simulink library "WECSim_Lib_Body_Elements"  (R2020b)
settings: Solver=VariableStepAuto  StartTime=0.0  StopTime=10.0  RelTol=1e-3
undefined symbols (not defined in the file or in its folder): body, simu, waves, X, Y, Z
libraries: nesl_utility x22, sm_lib x16, $bdroot x9, vrlib x3
(part 5 of 5)

== system WECSim_Lib_Body_Elements/Rigid Body/Hydrodynamic Body/Morison Element and Viscous Damping Force Calculation/Morison Element Variant Subsystem/Morison Element On/Regular Wave Morison Force ==
  displacement : Inport
  velocity : Inport  Port=2
  acceleration : Inport  Port=3
  time : Inport  Port=4
  Area : Constant  Value=body.morisonElement.area  VectorParams1D=off
  Ca : Constant  Value=body.morisonElement.ca  VectorParams1D=off
  Cd : Constant  Value=body.morisonElement.cd  VectorParams1D=off
  Current Depth : Constant  Value=waves.current.depth
  Current Direction : Constant  Value=waves.current.direction
  Current Option : Constant  Value=waves.current.option
  Current Speed : Constant  Value=waves.current.speed
  Density : Constant  Value=simu.rho
  Gravity : Constant  Value=simu.gravity
  MATLAB Function : MATLAB Function  TreatAsAtomicUnit=on
  Morison Element Option : Constant  Value=body.morisonElement.option
  Ramp Function Time : Constant  Value=simu.rampTime
  Volume : Constant  Value=body.morisonElement.VME  VectorParams1D=off
  WaterDepth : Constant  Value=waves.waterDepth
  WaveAmp : Constant  Value=waves.amplitude
  WaveFreq : Constant  Value=waves.omega
  WaveHeading : Constant  Value=waves.direction
  WaveNumber : Constant  Value=waves.wavenumber
  "r_{g}" : Constant  Value=body.morisonElement.rgME  VectorParams1D=off
  z : Constant  Value=body.morisonElement.z  VectorParams1D=off
  morison_force : Outport
  wires:
  MATLAB Function/1(f) -> morison_force/1
  z/1 -> MATLAB Function/1(z)
  Morison Element Option/1 -> MATLAB Function/23(simuMorison)
  Volume/1 -> MATLAB Function/8(Vol)
  velocity/1 -> MATLAB Function/3(Vel)
  Ramp Function Time/1 -> MATLAB Function/17(rampTime)
  "r_{g}"/1 -> MATLAB Function/2(r)
  time/1 -> MATLAB Function/10(Time)
  Current Depth/1 -> MATLAB Function/21(currentDepth)
  Current Option/1 -> MATLAB Function/22(currentOption)
  displacement/1 -> MATLAB Function/5(Disp)
  Cd/1 -> MATLAB Function/7(Cd)
  WaveFreq/1 -> MATLAB Function/15(w)
  WaveHeading/1 -> MATLAB Function/12(waveDir)
  Density/1 -> MATLAB Function/11(rho)
  acceleration/1 -> MATLAB Function/4(Accel)
  WaterDepth/1 -> MATLAB Function/13(waterDepth)
  Area/1 -> MATLAB Function/6(Area)
  Current Direction/1 -> MATLAB Function/20(currentDirection)
  Ca/1 -> MATLAB Function/9(Ca)
  WaveNumber/1 -> MATLAB Function/14(k)
  Gravity/1 -> MATLAB Function/18(g)
  WaveAmp/1 -> MATLAB Function/16(A)
  Current Speed/1 -> MATLAB Function/19(currentSpeed)

== system WECSim_Lib_Body_Elements/Rigid Body/Hydrodynamic Body/Wave Radiation Forces Calculation/SS CI and Constant-Damping-CoeVariant Subsystem/Convolution Integral Calculation/Convolution Variant Subsystem ==
  velocity : Inport
  Convolution Integral Calculation : Subsystem  VariantControl=sv_b1_noVariableHydro
  Convolution Integral Surface Calculation : Subsystem  VariantControl=sv_b1_variableHydro
  Frad : Outport

== system WECSim_Lib_Body_Elements/Rigid Body/Hydrodynamic Body/Wave Radiation Forces Calculation/SS CI and Constant-Damping-CoeVariant Subsystem/FIR Filter Calculation/FIR Filter Matrix ==
  velocity : Inport
  FIR_filter_row : Subsystem  mask{body=body, B2B=simu.b2b, rowNo=1}
      mask prompts: body "BodyClass"
      mask init: same as WECSim_Lib_Body_Elements/Flex Body/Wave Radiation Forces Calculation/Wave Radiation Forces Calculation/SS CI and Constant-Damping-CoeVariant Subsystem/FIR Filter Calculation/FIR Filter Matrix/FIR_filter_row
  Gain : Gain  Gain=simu.cicDt
  Mux : Mux  Inputs=1
  Out1 : Outport
  wires:
  Mux/1 -> Gain/1
  velocity/1 -> FIR_filter_row/1(In1)
  FIR_filter_row/1(Out1) -> Mux/1
  Gain/1 -> Out1/1

== system WECSim_Lib_Body_Elements/Flex Body/Wave Radiation Forces Calculation/Wave Radiation Forces Calculation/SS CI and Constant-Damping-CoeVariant Subsystem/Convolution Integral Calculation/Convolution Variant Subsystem/Convolution Integral Calculation ==
  note: Calculate the convolution integral using the radiation IRF (body.hydroForce.irkb) and the velocity.
  velocity : Inport
  Bus Selector : BusSelector  OutputSignals=irkb
  MATLAB Function : MATLAB Function  TreatAsAtomicUnit=on
  MATLAB Function1 : MATLAB Function  TreatAsAtomicUnit=on  SystemSampleTime=simu.cicDt
  Rate Transition : RateTransition  InitialCondition=simu.cicDt*[-1 -2 -3]
  Rate Transition1 : RateTransition
  cicTime : Constant  Value=simu.cicTime
  Frad : Outport
  wires:
  MATLAB Function1/2(FradExtrap) -> Rate Transition1/1
  MATLAB Function1/1(timeExtrap) -> Rate Transition/1
  Rate Transition/1 -> MATLAB Function/1(timeExtrap)
  Rate Transition1/1 -> MATLAB Function/2(FradExtrap)
  MATLAB Function/1(Frad) -> Frad/1
  [Clock] -> MATLAB Function1/4(time), MATLAB Function/3(time)
  velocity/1 -> MATLAB Function1/1(velocity)
  [body1_hydroForce] -> Bus Selector/1
  Bus Selector/1 -> MATLAB Function1/2(IRKB)  "<irkb>"
  cicTime/1 -> MATLAB Function1/3(cicTime)

== system WECSim_Lib_Body_Elements/Flex Body/Wave Radiation Forces Calculation/Wave Radiation Forces Calculation/SS CI and Constant-Damping-CoeVariant Subsystem/Convolution Integral Calculation/Convolution Variant Subsystem/Convolution Integral Surface Calculation ==
  note: Calculate the convolution integral using the radiation IRF surface (body.variableHydro.radiationIrfSurface) and the velocity.
  velocity : Inport
  MATLAB Function : MATLAB Function  TreatAsAtomicUnit=on
  Rate Transition : RateTransition  InitialCondition=simu.cicDt*[-1 -2 -3]
  Rate Transition1 : RateTransition
  cicTime : Constant  Value=simu.cicTime
  convolutionIntegralSurface : MATLAB Function  TreatAsAtomicUnit=on  SystemSampleTime=simu.cicDt
  hydroForceIndexInitial : Constant  Value=body.variableHydro.hydroForceIndexInitial
  radiationIrfSurface : Constant  Value=body.variableHydro.radiationIrfSurface
  Frad : Outport
  wires:
  Rate Transition/1 -> MATLAB Function/1(timeExtrap)
  Rate Transition1/1 -> MATLAB Function/2(FradExtrap)
  convolutionIntegralSurface/1(timeExtrap) -> Rate Transition/1
  convolutionIntegralSurface/2(FradExtrap) -> Rate Transition1/1
  MATLAB Function/1(Frad) -> Frad/1
  [Clock] -> convolutionIntegralSurface/6(time), MATLAB Function/3(time)
  [body1_hydroForce] -> convolutionIntegralSurface/2(hydroForceIndex)
  hydroForceIndexInitial/1 -> convolutionIntegralSurface/3(hydroForceIndexInitial)
  radiationIrfSurface/1 -> convolutionIntegralSurface/4(irkbSurfaceInput)
  cicTime/1 -> convolutionIntegralSurface/5(cicTime)
  velocity/1 -> convolutionIntegralSurface/1(velocity)

== system WECSim_Lib_Body_Elements/Flex Body/Wave Radiation Forces Calculation/Wave Radiation Forces Calculation/SS CI and Constant-Damping-CoeVariant Subsystem/FIR Filter Calculation/FIR Filter Matrix/FIR_filter_row ==
  In1 : Inport
  Add : Sum  Inputs=++++++
  Demux : Demux  Outputs=6
      settings: AttributesFormatString=%<Outputs>
  Discrete FIR Filter : DiscreteFir  Coefficients=transpose(squeeze(body.hydroForce.hf1.irkb(:,1,1)))
  Discrete FIR Filter 2 : DiscreteFir  Coefficients=transpose(squeeze(body.hydroForce.hf1.irkb(:,1,2)))
  Discrete FIR Filter 3 : DiscreteFir  Coefficients=transpose(squeeze(body.hydroForce.hf1.irkb(:,1,3)))
  Discrete FIR Filter 4 : DiscreteFir  Coefficients=transpose(squeeze(body.hydroForce.hf1.irkb(:,1,4)))
  Discrete FIR Filter 5 : DiscreteFir  Coefficients=transpose(squeeze(body.hydroForce.hf1.irkb(:,1,5)))
  Discrete FIR Filter 6 : DiscreteFir  Coefficients=transpose(squeeze(body.hydroForce.hf1.irkb(:,1,6)))
  Out1 : Outport
  wires:
  Discrete FIR Filter 6/1 -> Add/6
  Demux/6 -> Discrete FIR Filter 6/1
  Discrete FIR Filter 5/1 -> Add/5
  Demux/5 -> Discrete FIR Filter 5/1
  Discrete FIR Filter 4/1 -> Add/4
  Demux/4 -> Discrete FIR Filter 4/1
  Discrete FIR Filter 3/1 -> Add/3
  Demux/3 -> Discrete FIR Filter 3/1
  Discrete FIR Filter 2/1 -> Add/2
  Demux/2 -> Discrete FIR Filter 2/1
  Discrete FIR Filter/1 -> Add/1
  Demux/1 -> Discrete FIR Filter/1
  Add/1 -> Out1/1
  In1/1 -> Demux/1

== system WECSim_Lib_Body_Elements/Rigid Body/Hydrodynamic Body/Wave Radiation Forces Calculation/SS CI and Constant-Damping-CoeVariant Subsystem/Convolution Integral Calculation/Convolution Variant Subsystem/Convolution Integral Calculation ==
  note: Calculate the convolution integral using the radiation IRF (body.hydroForce.irkb) and the velocity.
  velocity : Inport
  Bus Selector : BusSelector  OutputSignals=irkb
  MATLAB Function : MATLAB Function  TreatAsAtomicUnit=on
  MATLAB Function1 : MATLAB Function  TreatAsAtomicUnit=on  SystemSampleTime=simu.cicDt
  Rate Transition : RateTransition  InitialCondition=simu.cicDt*[-1 -2 -3]
  Rate Transition1 : RateTransition
  cicTime : Constant  Value=simu.cicTime
  Frad : Outport
  wires:
  cicTime/1 -> MATLAB Function1/3(cicTime)
  Bus Selector/1 -> MATLAB Function1/2(IRKB)  "<irkb>"
  [body1_hydroForce] -> Bus Selector/1
  velocity/1 -> MATLAB Function1/1(velocity)
  [Clock] -> MATLAB Function/3(time), MATLAB Function1/4(time)
  MATLAB Function/1(Frad) -> Frad/1
  Rate Transition1/1 -> MATLAB Function/2(FradExtrap)
  Rate Transition/1 -> MATLAB Function/1(timeExtrap)
  MATLAB Function1/1(timeExtrap) -> Rate Transition/1
  MATLAB Function1/2(FradExtrap) -> Rate Transition1/1

== system WECSim_Lib_Body_Elements/Rigid Body/Hydrodynamic Body/Wave Radiation Forces Calculation/SS CI and Constant-Damping-CoeVariant Subsystem/Convolution Integral Calculation/Convolution Variant Subsystem/Convolution Integral Surface Calculation ==
  note: Calculate the convolution integral using the radiation IRF surface (body.variableHydro.radiationIrfSurface) and the velocity.
  velocity : Inport
  MATLAB Function : MATLAB Function  TreatAsAtomicUnit=on
  Rate Transition : RateTransition  InitialCondition=simu.cicDt*[-1 -2 -3]
  Rate Transition1 : RateTransition
  cicTime : Constant  Value=simu.cicTime
  convolutionIntegralSurface : MATLAB Function  TreatAsAtomicUnit=on  SystemSampleTime=simu.cicDt
  hydroForceIndexInitial : Constant  Value=body.variableHydro.hydroForceIndexInitial
  radiationIrfSurface : Constant  Value=body.variableHydro.radiationIrfSurface
  Frad : Outport
  wires:
  velocity/1 -> convolutionIntegralSurface/1(velocity)
  cicTime/1 -> convolutionIntegralSurface/5(cicTime)
  radiationIrfSurface/1 -> convolutionIntegralSurface/4(irkbSurfaceInput)
  hydroForceIndexInitial/1 -> convolutionIntegralSurface/3(hydroForceIndexInitial)
  [body1_hydroForceIndex] -> convolutionIntegralSurface/2(hydroForceIndex)
  [Clock] -> MATLAB Function/3(time), convolutionIntegralSurface/6(time)
  MATLAB Function/1(Frad) -> Frad/1
  convolutionIntegralSurface/2(FradExtrap) -> Rate Transition1/1
  convolutionIntegralSurface/1(timeExtrap) -> Rate Transition/1
  Rate Transition1/1 -> MATLAB Function/2(FradExtrap)
  Rate Transition/1 -> MATLAB Function/1(timeExtrap)

== system WECSim_Lib_Body_Elements/Rigid Body/Hydrodynamic Body/Wave Radiation Forces Calculation/SS CI and Constant-Damping-CoeVariant Subsystem/FIR Filter Calculation/FIR Filter Matrix/FIR_filter_row ==
  In1 : Inport
  Add : Sum  Inputs=++++++
  Demux : Demux  Outputs=6
      settings: AttributesFormatString=%<Outputs>
  Discrete FIR Filter : DiscreteFir  Coefficients=transpose(squeeze(body.hydroForce.hf1.irkb(:,1,1)))
  Discrete FIR Filter 2 : DiscreteFir  Coefficients=transpose(squeeze(body.hydroForce.hf1.irkb(:,1,2)))
  Discrete FIR Filter 3 : DiscreteFir  Coefficients=transpose(squeeze(body.hydroForce.hf1.irkb(:,1,3)))
  Discrete FIR Filter 4 : DiscreteFir  Coefficients=transpose(squeeze(body.hydroForce.hf1.irkb(:,1,4)))
  Discrete FIR Filter 5 : DiscreteFir  Coefficients=transpose(squeeze(body.hydroForce.hf1.irkb(:,1,5)))
  Discrete FIR Filter 6 : DiscreteFir  Coefficients=transpose(squeeze(body.hydroForce.hf1.irkb(:,1,6)))
  Out1 : Outport
  wires:
  In1/1 -> Demux/1
  Add/1 -> Out1/1
  Demux/1 -> Discrete FIR Filter/1
  Discrete FIR Filter/1 -> Add/1
  Demux/2 -> Discrete FIR Filter 2/1
  Discrete FIR Filter 2/1 -> Add/2
  Demux/3 -> Discrete FIR Filter 3/1
  Discrete FIR Filter 3/1 -> Add/3
  Demux/4 -> Discrete FIR Filter 4/1
  Discrete FIR Filter 4/1 -> Add/4
  Demux/5 -> Discrete FIR Filter 5/1
  Discrete FIR Filter 5/1 -> Add/5
  Demux/6 -> Discrete FIR Filter 6/1
  Discrete FIR Filter 6/1 -> Add/6

== matlab function WECSim_Lib_Body_Elements/Rigid Body/Hydrodynamic Body/Morison Element and Viscous Damping Force Calculation/Morison Element Variant Subsystem/Morison Element On/No Wave Morison Force/MorisonElement(s) ==
  data: z input; f output; r input; Vel input; Accel input; Disp input; Area input; Cd input; Vol input; Ca input; Time input; rho input; rampTime input; currentSpeed input; currentDirection input; currentDepth input; currentOption input; bodyMorison input
function f = noWaveMorison(z,r,Vel,Accel,Disp,Area,Cd,Vol,Ca,Time,rho,rampTime,currentSpeed,currentDirection,currentDepth,currentOption,bodyMorison)

f = noWaveMorison(z,r,Vel,Accel,Disp,Area,Cd,Vol,Ca,Time,rho,rampTime,currentSpeed,currentDirection,currentDepth,currentOption,bodyMorison);

end

== matlab function WECSim_Lib_Body_Elements/Rigid Body/Hydrodynamic Body/Morison Element and Viscous Damping Force Calculation/Morison Element Variant Subsystem/Morison Element On/Irregular Wave Morison Force/MATLAB Function ==
  data: z input; f output; r input; Vel input; Accel input; Disp input; Area input; Cd input; Vol input; Ca input; Time input; rho input; waveDir input; waveSpread input; waterDepth input; k input; w input; A input; rampTime input; g input; randPhase input; dw input; currentSpeed input; currentDirection input; currentDepth input; currentOption input; simuMorison input
function f = irregWaveMorison(z,r,Vel,Accel,Disp,Area,Cd,Vol,Ca,Time,rho,waveDir,waveSpread,waterDepth,k,w,A,rampTime,g,randPhase,dw,currentSpeed,currentDirection,currentDepth,currentOption,simuMorison)

f = irregWaveMorison(z,r,Vel,Accel,Disp,Area,Cd,Vol,Ca,Time,rho,waveDir,waveSpread,waterDepth,k,w,A,rampTime,g,randPhase,dw,currentSpeed,currentDirection,currentDepth,currentOption,simuMorison);

end

== matlab function WECSim_Lib_Body_Elements/Rigid Body/Hydrodynamic Body/Wave Diffraction and Excitation Force Calculation/Linear Wave Excitation Force Variant Subsystem/Irregular Wave Excitation Force/MATLAB Function2 ==
  data: disp input; dispPhase output; enable input; frequency input; wavenumber input; direction input
function dispPhase  = calcDispPhase(disp, enable, frequency, wavenumber, direction)
% initialize
dispPhase = zeros(length(frequency),length(direction));
% execute
dispPhase = calcDispPhase(disp, enable, direction, frequency, wavenumber);

end

== matlab function WECSim_Lib_Body_Elements/Rigid Body/Hydrodynamic Body/Wave Diffraction and Excitation Force Calculation/Linear Wave Excitation Force Variant Subsystem/Regular Wave NonLinear Yaw/MATLAB Function3 ==
  data: disp input; dispPhase output; enable input; frequency input; wavenumber input; direction input
function dispPhase  = calcDispPhase(disp, enable, frequency, wavenumber, direction)
% initialize
dispPhase = zeros(length(frequency),length(direction));
% execute
dispPhase = calcDispPhase(disp, enable, direction, frequency, wavenumber);

end

== matlab function WECSim_Lib_Body_Elements/Rigid Body/Hydrodynamic Body/Wave Radiation Forces Calculation/SS CI and Constant-Damping-CoeVariant Subsystem/Convolution Integral Calculation/Convolution Variant Subsystem/Convolution Integral Surface Calculation/convolutionIntegralSurface ==
  data: velocity input; timeExtrap output; hydroForceIndex input; hydroForceIndexInitial input; irkbSurfaceInput input; cicTime input; time input; FradExtrap output
function [timeExtrap, FradExtrap] = convolutionIntegralSurface(velocity, hydroForceIndex, hydroForceIndexInitial, irkbSurfaceInput, cicTime, time)

[timeExtrap, FradExtrap] = convolutionIntegralSurface(velocity, hydroForceIndex, hydroForceIndexInitial, irkbSurfaceInput, cicTime, time);

end

== matlab function WECSim_Lib_Body_Elements/Rigid Body/Hydrodynamic Body/Wave Diffraction and Excitation Force Calculation/Linear Wave Excitation Force Variant Subsystem/Regular Wave Excitation Force/MATLAB Function1 ==
  data: disp input; dispPhase output; enable input; frequency input; wavenumber input; direction input
function dispPhase  = calcDispPhase(disp, enable, frequency, wavenumber, direction)
% initialize
dispPhase = zeros(length(frequency),length(direction));
% execute
dispPhase = calcDispPhase(disp, enable, direction, frequency, wavenumber);

end

== matlab function WECSim_Lib_Body_Elements/Rigid Body/Hydrodynamic Body/Wave Radiation Forces Calculation/SS CI and Constant-Damping-CoeVariant Subsystem/Convolution Integral Calculation/Convolution Variant Subsystem/Convolution Integral Surface Calculation/MATLAB Function ==
  data: timeExtrap input; FradExtrap input; time input; Frad output
function Frad =  extrapFrad(timeExtrap, FradExtrap, time)

Frad =  extrapFrad(timeExtrap, FradExtrap, time);

end

== matlab function WECSim_Lib_Body_Elements/Flex Body/Wave Radiation Forces Calculation/Wave Radiation Forces Calculation/SS CI and Constant-Damping-CoeVariant Subsystem/Convolution Integral Calculation/Convolution Variant Subsystem/Convolution Integral Calculation/MATLAB Function ==
  data: timeExtrap input; FradExtrap input; time input; Frad output
function Frad =  extrapFrad(timeExtrap, FradExtrap, time)

Frad =  extrapFrad(timeExtrap, FradExtrap, time);

end

== matlab function WECSim_Lib_Body_Elements/Rigid Body/Hydrodynamic Body/Nonlinear Wave Elevation/Linear or Instantaneous Free Surface/Instantaneous Water Free Surface/Instantaneous FS ==
  data: x input; center input; f output; cg input; AH input; w input; dw input; k input; typeNum input; t input; rampT input; phaseRand input; waveDir input; spread input
function f  = waveElevation(x,center,cg,AH,w,dw,k,typeNum,t,rampT,phaseRand,waveDir,spread)

f  = waveElevation(x,center,cg,AH,w,dw,k,typeNum,t,rampT,phaseRand,waveDir,spread);

end

== matlab function WECSim_Lib_Body_Elements/Rigid Body/Hydrodynamic Body/Structure/Motion Sensor/quaternion2EulXYZ ==
  data: Q input; E output
function E = quaternion2EulXYZ(Q)

E = quaternion2EulXYZ(Q);

end

== matlab function WECSim_Lib_Body_Elements/Rigid Body/Hydrodynamic Body/Wave Diffraction and Excitation Force Calculation/Linear Wave Excitation Force Variant Subsystem/Irregular Wave Excitation Force/MATLAB Function ==
  data: A input; Fext output; w input; fExtRE input; fExtIM input; phaseRand input; dw input; time input; WaveDir input; spread input; fExtMD input
function Fext = irregExcF(A,w,fExtRE,fExtIM,phaseRand,dw,time,WaveDir,spread,fExtMD)

Fext = irregExcF(A,w,fExtRE,fExtIM,phaseRand,dw,time,WaveDir,spread,fExtMD);

end

== matlab function WECSim_Lib_Body_Elements/Rigid Body/Hydrodynamic Body/Wave Diffraction and Excitation Force Calculation/Nonlinear FK Force Variant Subsystem/With Nonlinear FroudeKrylov Force/Diffraction and Excitation Forces ==
  data: x input; elv input; direction input; spread input; center input; f output; tnorm input; area input; rho input; g input; cg input; AH input; w input; dw input; wDepth input; deepWater input; k input; typeNum input; t input; phaseRand input; wp output; wpMeanFS output
function [f, wp, wpMeanFS]  = nonFKForce(x,elv,direction,spread,center,tnorm,area,rho,g,cg,AH,w,dw,wDepth,deepWater,k,typeNum,t,phaseRand)

[f, wp, wpMeanFS]  = nonFKForce(x,elv,direction,spread,center,tnorm,area,rho,g,cg,AH,w,dw,wDepth,deepWater,k,typeNum,t,phaseRand);

end

== matlab function WECSim_Lib_Body_Elements/Rigid Body/Hydrodynamic Body/Wave Radiation Forces Calculation/SS CI and Constant-Damping-CoeVariant Subsystem/Convolution Integral Calculation/Convolution Variant Subsystem/Convolution Integral Calculation/MATLAB Function1 ==
  data: velocity input; timeExtrap output; IRKB input; cicTime input; FradExtrap output; time input
function [timeExtrap, FradExtrap] = convolutionIntegralInterp(velocity, IRKB, cicTime, time)

[timeExtrap, FradExtrap] = convolutionIntegralInterp(velocity, IRKB, cicTime, time);

end

== matlab function WECSim_Lib_Body_Elements/Flex Body/Wave Diffraction and Excitation Force Calculation/Wave Diffraction and Excitation Force Calculation/Linear Wave Excitation Force Variant Subsystem/Regular Wave Excitation Force/MATLAB Function1 ==
  data: disp input; dispPhase output; enable input; frequency input; wavenumber input; direction input
function dispPhase  = calcDispPhase(disp, enable, frequency, wavenumber, direction)
% initialize
dispPhase = zeros(length(frequency),length(direction));
% execute
dispPhase = calcDispPhase(disp, enable, direction, frequency, wavenumber);

end

== matlab function WECSim_Lib_Body_Elements/Rigid Body/Hydrodynamic Body/Yaw Force Transforms/Yaw Force Transforms ==
  data: yaw input; F_Excitation output; dispGlobal input; F_RadiationDampingLocal input; F_AddedMassLocal input; F_ExcitationLocal input; F_RadiationDamping output; F_RestoringLocal input; F_AddedMass output; F_Restoring output
function [F_Excitation, F_RadiationDamping, F_AddedMass, F_Restoring] = fYawTransforms(yaw, dispGlobal, F_RadiationDampingLocal, F_AddedMassLocal, F_ExcitationLocal, F_RestoringLocal)

[F_Excitation, F_RadiationDamping, F_AddedMass, F_Restoring] = fYawTransforms(yaw, dispGlobal, F_RadiationDampingLocal, F_AddedMassLocal, F_ExcitationLocal, F_RestoringLocal);

end

== matlab function WECSim_Lib_Body_Elements/Rigid Body/Hydrodynamic Body/Wave Diffraction and Excitation Force Calculation/Linear Wave Excitation Force Variant Subsystem/Regular Wave NonLinear Yaw/MATLAB Function1 ==
  data: A input; w input; dofGRD input; dirGRD input; fEHRE input; fEHIM input; Fext output; fEHMD input; time input; WaveDir input; Disp input; intThresh input; phase input; prevYaw input; relYawLast output; prevCoeffMD input; prevCoeffRE input; prevCoeffIM input; coeffsLastMD output; coeffsLastRE output; coeffsLastIM output
function [Fext,relYawLast,coeffsLastMD,coeffsLastRE,coeffsLastIM] = regnLYaw(A,w,dofGRD,dirGRD,fEHRE,fEHIM, fEHMD,time,WaveDir,Disp, intThresh, phase, prevYaw, prevCoeffMD, prevCoeffRE, prevCoeffIM)

%initialize outputs
Fext = zeros(1,6);
relYawLast=0;
coeffsLastMD=zeros(length(w),6); 
coeffsLastRE=zeros(length(w),6);
coeffsLastIM=zeros(length(w),6);

[Fext,relYawLast,coeffsLastMD,coeffsLastRE,coeffsLastIM] = regnLYaw(A,w,dofGRD,dirGRD,fEHRE,fEHIM, fEHMD,time,WaveDir,Disp, intThresh, phase, prevYaw, prevCoeffMD, prevCoeffRE, prevCoeffIM);

end

== matlab function WECSim_Lib_Body_Elements/Rigid Body/Hydrodynamic Body/Yaw Kinematic Transforms/No B2B/Yaw Kinematic Transforms ==
  data: yaw input; dispLoc output; dispGlobal input; velGlobal input; accGlobal input; velLoc output; accLoc output
function [dispLoc, velLoc, accLoc] = kinYawTransform(yaw, dispGlobal, velGlobal, accGlobal)

[dispLoc, velLoc, accLoc] = kinYawTransformNoB2B(yaw, dispGlobal, velGlobal, accGlobal);

end

== matlab function WECSim_Lib_Body_Elements/Rigid Body/Hydrodynamic Body/Wave Diffraction and Excitation Force Calculation/Second Order Excitation Force Variant Subsystem/With Second Order Excitation Force/Diffraction and Excitation Forces ==
  data: time_vector input; fastVaryingForce input; f output; slowVaryingForce input; t input; displacement input
function f   = secondOrderExt(time_vector, fastVaryingForce, slowVaryingForce, t, displacement)

f  = secondOrderExt(time_vector, fastVaryingForce, slowVaryingForce, t, displacement);

end

== matlab function WECSim_Lib_Body_Elements/Flex Body/Wave Diffraction and Excitation Force Calculation/Wave Diffraction and Excitation Force Calculation/Nonlinear FK Force Variant Subsystem/With Nonlinear FroudeKrylov Force/Diffraction and Excitation Forces ==
  data: x input; elv input; direction input; spread input; center input; f output; tnorm input; area input; rho input; g input; cg input; AH input; w input; dw input; wDepth input; deepWater input; k input; typeNum input; t input; phaseRand input; wp output; wpMeanFS output
function [f, wp, wpMeanFS]  = nonFKForce(x,elv,direction,spread,center,tnorm,area,rho,g,cg,AH,w,dw,wDepth,deepWater,k,typeNum,t,phaseRand)

[f, wp, wpMeanFS]  = nonFKForce(x,elv,direction,spread,center,tnorm,area,rho,g,cg,AH,w,dw,wDepth,deepWater,k,typeNum,t,phaseRand);

end

== matlab function WECSim_Lib_Body_Elements/Rigid Body/Hydrodynamic Body/Yaw Kinematic Transforms/With B2B/Yaw Kinematic Transforms ==
  data: yaw input; dispLoc output; dispGlobal input; velGlobal input; accGlobal input; velLoc output; accLoc output; numBody parameter
function [dispLoc, velLoc, accLoc] = kinYawTransformB2B(yaw, dispGlobal, velGlobal, accGlobal, numBody)

[dispLoc, velLoc, accLoc] = kinYawTransformB2B(yaw, dispGlobal, velGlobal, accGlobal, numBody);

end

== matlab function WECSim_Lib_Body_Elements/Rigid Body/Hydrodynamic Body/Morison Element and Viscous Damping Force Calculation/Morison Element Variant Subsystem/Morison Element On/Regular Wave Morison Force/MATLAB Function ==
  data: z input; f output; r input; Vel input; Accel input; Disp input; Area input; Cd input; Vol input; Ca input; Time input; rho input; waveDir input; waterDepth input; k input; w input; A input; rampTime input; g input; currentSpeed input; currentDirection input; currentDepth input; currentOption input; simuMorison input
function f = regWaveMorison(z,r,Vel,Accel,Disp,Area,Cd,Vol,Ca,Time,rho,waveDir,waterDepth,k,w,A,rampTime,g,currentSpeed,currentDirection,currentDepth,currentOption,simuMorison)

f = regWaveMorison(z,r,Vel,Accel,Disp,Area,Cd,Vol,Ca,Time,rho,waveDir,waterDepth,k,w,A,rampTime,g,currentSpeed,currentDirection,currentDepth,currentOption,simuMorison);

end

== matlab function WECSim_Lib_Body_Elements/Flex Body/Wave Radiation Forces Calculation/Wave Radiation Forces Calculation/SS CI and Constant-Damping-CoeVariant Subsystem/Convolution Integral Calculation/Convolution Variant Subsystem/Convolution Integral Calculation/MATLAB Function1 ==
  data: velocity input; timeExtrap output; IRKB input; cicTime input; FradExtrap output; time input
function [timeExtrap, FradExtrap] = convolutionIntegralInterp(velocity, IRKB, cicTime, time)

[timeExtrap, FradExtrap] = convolutionIntegralInterp(velocity, IRKB, cicTime, time);

end

== matlab function WECSim_Lib_Body_Elements/Flex Body/Wave Radiation Forces Calculation/Wave Radiation Forces Calculation/SS CI and Constant-Damping-CoeVariant Subsystem/Convolution Integral Calculation/Convolution Variant Subsystem/Convolution Integral Surface Calculation/MATLAB Function ==
  data: timeExtrap input; FradExtrap input; time input; Frad output
function Frad =  extrapFrad(timeExtrap, FradExtrap, time)

Frad =  extrapFrad(timeExtrap, FradExtrap, time);

end

== matlab function WECSim_Lib_Body_Elements/Flex Body/Wave Radiation Forces Calculation/Wave Radiation Forces Calculation/SS CI and Constant-Damping-CoeVariant Subsystem/Convolution Integral Calculation/Convolution Variant Subsystem/Convolution Integral Surface Calculation/convolutionIntegralSurface ==
  data: velocity input; timeExtrap output; hydroForceIndex input; hydroForceIndexInitial input; irkbSurfaceInput input; cicTime input; time input; FradExtrap output
function [timeExtrap, FradExtrap] = convolutionIntegralSurface(velocity, hydroForceIndex, hydroForceIndexInitial, irkbSurfaceInput, cicTime, time)

[timeExtrap, FradExtrap] = convolutionIntegralSurface(velocity, hydroForceIndex, hydroForceIndexInitial, irkbSurfaceInput, cicTime, time);

end

== matlab function WECSim_Lib_Body_Elements/Rigid Body/Hydrodynamic Body/Wave Diffraction and Excitation Force Calculation/Linear Wave Excitation Force Variant Subsystem/Irregular Wave NonLinearYaw/MATLAB Function1 ==
  data: disp input; dispPhase output; enable input; frequency input; wavenumber input; direction input
function dispPhase  = calcDispPhase(disp, enable, frequency, wavenumber, direction)
% initialize
dispPhase = zeros(length(frequency),length(direction));
% execute
dispPhase = calcDispPhase(disp, enable, direction, frequency, wavenumber);

end

== matlab function WECSim_Lib_Body_Elements/Flex Body/Wave Diffraction and Excitation Force Calculation/Wave Diffraction and Excitation Force Calculation/Linear Wave Excitation Force Variant Subsystem/Irregular Wave Full Direction/MATLAB Function ==
  data: passiveYaw input; amplitude input; omega input; dofGRD input; dirGRD input; wGRD input; qDofGRD input; qWGRD input; fEHRE input; fEHIM input; fEHMD input; phaseRand input; dOmega input; time input; directions input; Fext output; relYawLast output; disp input; yawThresh input; prevYaw input; prevCoeffMD input; prevCoeffRE input; prevCoeffIM input; coeffsLastMD output; coeffsLastRE output; coeffsLastIM output
function [Fext, relYawLast, coeffsLastMD,coeffsLastRE,coeffsLastIM] = irregExcFullDirF(passiveYaw, amplitude, omega, dofGRD, dirGRD, wGRD, qDofGRD, qWGRD, fEHRE, fEHIM, fEHMD, phaseRand, dOmega, time, directions, disp, yawThresh, prevYaw, prevCoeffMD, prevCoeffRE, prevCoeffIM)

[Fext,relYawLast,coeffsLastMD,coeffsLastRE,coeffsLastIM] = irregExcFullDirF(passiveYaw, amplitude, omega, dofGRD, dirGRD, wGRD, qDofGRD, qWGRD, fEHRE, fEHIM, fEHMD, phaseRand, dOmega, time, directions, disp, yawThresh, prevYaw, prevCoeffMD, prevCoeffRE, prevCoeffIM);

end

== matlab function WECSim_Lib_Body_Elements/Rigid Body/Hydrodynamic Body/Hydrostatic Restoring Force Calculation/Linear and Nonlinear Restoring Force Variant Subsystem/Nonlinear Hydrostatic Restoring Force/Restoring Forces ==
  data: x input; elv input; center input; f output; tnorm input; area input; rho input; g input; cg input; p output; mass input
function [f,p]  = nonLinearBuoyancy(x,elv,center,tnorm,area,rho,g,cg,mass)

[f,p]  = nonLinearBuoyancy(x,elv,center,tnorm,area,rho,g,cg,mass);

end

== matlab function WECSim_Lib_Body_Elements/Rigid Body/Hydrodynamic Body/Wave Diffraction and Excitation Force Calculation/Linear Wave Excitation Force Variant Subsystem/Irregular Wave Full Direction/MATLAB Function ==
  data: passiveYaw input; amplitude input; omega input; dofGRD input; dirGRD input; wGRD input; qDofGRD input; qWGRD input; fEHRE input; fEHIM input; fEHMD input; phaseRand input; dOmega input; time input; directions input; Fext output; relYawLast output; disp input; yawThresh input; prevYaw input; prevCoeffMD input; prevCoeffRE input; prevCoeffIM input; coeffsLastMD output; coeffsLastRE output; coeffsLastIM output
function [Fext, relYawLast, coeffsLastMD,coeffsLastRE,coeffsLastIM] = irregExcFullDirF(passiveYaw, amplitude, omega, dofGRD, dirGRD, wGRD, qDofGRD, qWGRD, fEHRE, fEHIM, fEHMD, phaseRand, dOmega, time, directions, disp, yawThresh, prevYaw, prevCoeffMD, prevCoeffRE, prevCoeffIM)

[Fext,relYawLast,coeffsLastMD,coeffsLastRE,coeffsLastIM] = irregExcFullDirF(passiveYaw, amplitude, omega, dofGRD, dirGRD, wGRD, qDofGRD, qWGRD, fEHRE, fEHIM, fEHMD, phaseRand, dOmega, time, directions, disp, yawThresh, prevYaw, prevCoeffMD, prevCoeffRE, prevCoeffIM);

end

== matlab function WECSim_Lib_Body_Elements/Rigid Body/Hydrodynamic Body/Wave Diffraction and Excitation Force Calculation/Linear Wave Excitation Force Variant Subsystem/Irregular Wave Full Direction/MATLAB Function1 ==
  data: disp input; dispPhase output; enable input; frequency input; wavenumber input; directions input
function dispPhase  = calcDispPhase(disp, enable, frequency, wavenumber, directions)
% initialize
dispPhase = zeros(length(frequency),length(directions));
% execute
dispPhase = calcDispPhase(disp, enable, directions, frequency, wavenumber);

end

== matlab function WECSim_Lib_Body_Elements/Flex Body/Wave Diffraction and Excitation Force Calculation/Wave Diffraction and Excitation Force Calculation/Linear Wave Excitation Force Variant Subsystem/Irregular Wave Full Direction/MATLAB Function1 ==
  data: disp input; dispPhase output; enable input; frequency input; wavenumber input; directions input
function dispPhase  = calcDispPhase(disp, enable, frequency, wavenumber, directions)
% initialize
dispPhase = zeros(length(frequency),length(directions));
% execute
dispPhase = calcDispPhase(disp, enable, directions, frequency, wavenumber);

end

== matlab function WECSim_Lib_Body_Elements/Flex Body/Wave Diffraction and Excitation Force Calculation/Wave Diffraction and Excitation Force Calculation/Linear Wave Excitation Force Variant Subsystem/Regular Wave NonLinear Yaw/MATLAB Function1 ==
  data: A input; w input; dofGRD input; dirGRD input; fEHRE input; fEHIM input; Fext output; fEHMD input; time input; WaveDir input; Disp input; intThresh input; phase input; prevYaw input; relYawLast output; prevCoeffMD input; prevCoeffRE input; prevCoeffIM input; coeffsLastMD output; coeffsLastRE output; coeffsLastIM output
function [Fext,relYawLast,coeffsLastMD,coeffsLastRE,coeffsLastIM] = regnLYaw(A,w,dofGRD,dirGRD,fEHRE,fEHIM, fEHMD,time,WaveDir,Disp, intThresh, phase, prevYaw, prevCoeffMD, prevCoeffRE, prevCoeffIM)

%initialize outputs
Fext = zeros(1,6);
relYawLast=0;
coeffsLastMD=zeros(length(w),6); 
coeffsLastRE=zeros(length(w),6);
coeffsLastIM=zeros(length(w),6);

[Fext,relYawLast,coeffsLastMD,coeffsLastRE,coeffsLastIM] = regnLYaw(A,w,dofGRD,dirGRD,fEHRE,fEHIM, fEHMD,time,WaveDir,Disp, intThresh, phase, prevYaw, prevCoeffMD, prevCoeffRE, prevCoeffIM);

end

== matlab function WECSim_Lib_Body_Elements/Flex Body/Wave Diffraction and Excitation Force Calculation/Wave Diffraction and Excitation Force Calculation/Linear Wave Excitation Force Variant Subsystem/Regular Wave NonLinear Yaw/MATLAB Function3 ==
  data: disp input; dispPhase output; enable input; frequency input; wavenumber input; direction input
function dispPhase  = calcDispPhase(disp, enable, frequency, wavenumber, direction)
% initialize
dispPhase = zeros(length(frequency),length(direction));
% execute
dispPhase = calcDispPhase(disp, enable, direction, frequency, wavenumber);

end

== matlab function WECSim_Lib_Body_Elements/Flex Body/Wave Diffraction and Excitation Force Calculation/Wave Diffraction and Excitation Force Calculation/Linear Wave Excitation Force Variant Subsystem/Irregular Wave Excitation Force/MATLAB Function ==
  data: A input; Fext output; w input; fExtRE input; fExtIM input; phaseRand input; dw input; time input; WaveDir input; spread input; fExtMD input
function Fext = irregExcF(A,w,fExtRE,fExtIM,phaseRand,dw,time,WaveDir,spread,fExtMD)

Fext = irregExcF(A,w,fExtRE,fExtIM,phaseRand,dw,time,WaveDir,spread,fExtMD);

end

== matlab function WECSim_Lib_Body_Elements/Flex Body/Wave Diffraction and Excitation Force Calculation/Wave Diffraction and Excitation Force Calculation/Linear Wave Excitation Force Variant Subsystem/Irregular Wave Excitation Force/MATLAB Function2 ==
  data: disp input; dispPhase output; enable input; frequency input; wavenumber input; direction input
function dispPhase  = calcDispPhase(disp, enable, frequency, wavenumber, direction)
% initialize
dispPhase = zeros(length(frequency),length(direction));
% execute
dispPhase = calcDispPhase(disp, enable, direction, frequency, wavenumber);

end

== matlab function WECSim_Lib_Body_Elements/Flex Body/Wave Diffraction and Excitation Force Calculation/Wave Diffraction and Excitation Force Calculation/Linear Wave Excitation Force Variant Subsystem/Irregular Wave NonLinearYaw/MATLAB Function ==
  data: A input; w input; dofGRD input; dirGRD input; wGRD input; fEHRE input; fEHIM input; Fext output; fEHMD input; phaseRand input; dw input; time input; direction input; spread input; Disp input; intThresh input; prevYaw input; relYawLast output; prevCoeffMD input; prevCoeffRE input; prevCoeffIM input; coeffsLastMD output; coeffsLastRE output; coeffsLastIM output
function [Fext,relYawLast,coeffsLastMD,coeffsLastRE,coeffsLastIM] = irregnLYaw(A,w,dofGRD,dirGRD,wGRD,fEHRE,fEHIM, fEHMD, phaseRand,dw,time,direction,spread, Disp, intThresh, prevYaw, prevCoeffMD, prevCoeffRE, prevCoeffIM)

%initialize outputs
Fext = zeros(1,6);
relYawLast=0;
coeffsLastMD=zeros(length(w),6);
coeffsLastRE=zeros(length(w),6);
coeffsLastIM=zeros(length(w),6);

[Fext,relYawLast,coeffsLastMD,coeffsLastRE,coeffsLastIM] = irregnLYaw(A,w,dofGRD,dirGRD,wGRD,fEHRE,fEHIM, fEHMD, phaseRand,dw,time,direction,spread, Disp, intThresh, prevYaw, prevCoeffMD, prevCoeffRE, prevCoeffIM);

end

== matlab function WECSim_Lib_Body_Elements/Flex Body/Hydrostatic Restoring Force Calculation/Hydrostatic Restoring Force Calculation/Linear and Nonlinear Restoring Force Variant Subsystem/Nonlinear Hydrostatic Restoring Force/Restoring Forces ==
  data: x input; elv input; center input; f output; tnorm input; area input; rho input; g input; cg input; p output; mass input
function [f,p]  = nonLinearBuoyancy(x,elv,center,tnorm,area,rho,g,cg,mass)

[f,p]  = nonLinearBuoyancy(x,elv,center,tnorm,area,rho,g,cg,mass);

end

== matlab function WECSim_Lib_Body_Elements/Flex Body/Wave Diffraction and Excitation Force Calculation/Wave Diffraction and Excitation Force Calculation/Linear Wave Excitation Force Variant Subsystem/Irregular Wave NonLinearYaw/MATLAB Function1 ==
  data: disp input; dispPhase output; enable input; frequency input; wavenumber input; direction input
function dispPhase  = calcDispPhase(disp, enable, frequency, wavenumber, direction)
% initialize
dispPhase = zeros(length(frequency),length(direction));
% execute
dispPhase = calcDispPhase(disp, enable, direction, frequency, wavenumber);

end

== matlab function WECSim_Lib_Body_Elements/Rigid Body/Hydrodynamic Body/Wave Radiation Forces Calculation/SS CI and Constant-Damping-CoeVariant Subsystem/Convolution Integral Calculation/Convolution Variant Subsystem/Convolution Integral Calculation/MATLAB Function ==
  data: timeExtrap input; FradExtrap input; time input; Frad output
function Frad =  extrapFrad(timeExtrap, FradExtrap, time)

Frad =  extrapFrad(timeExtrap, FradExtrap, time);

end

== matlab function WECSim_Lib_Body_Elements/Rigid Body/Hydrodynamic Body/Wave Diffraction and Excitation Force Calculation/Linear Wave Excitation Force Variant Subsystem/Irregular Wave NonLinearYaw/MATLAB Function ==
  data: A input; w input; dofGRD input; dirGRD input; wGRD input; fEHRE input; fEHIM input; Fext output; fEHMD input; phaseRand input; dw input; time input; direction input; spread input; Disp input; intThresh input; prevYaw input; relYawLast output; prevCoeffMD input; prevCoeffRE input; prevCoeffIM input; coeffsLastMD output; coeffsLastRE output; coeffsLastIM output
function [Fext,relYawLast,coeffsLastMD,coeffsLastRE,coeffsLastIM] = irregnLYaw(A,w,dofGRD,dirGRD,wGRD,fEHRE,fEHIM, fEHMD, phaseRand,dw,time,direction,spread, Disp, intThresh, prevYaw, prevCoeffMD, prevCoeffRE, prevCoeffIM)

%initialize outputs
Fext = zeros(1,6);
relYawLast=0;
coeffsLastMD=zeros(length(w),6);
coeffsLastRE=zeros(length(w),6);
coeffsLastIM=zeros(length(w),6);

[Fext,relYawLast,coeffsLastMD,coeffsLastRE,coeffsLastIM] = irregnLYaw(A,w,dofGRD,dirGRD,wGRD,fEHRE,fEHIM, fEHMD, phaseRand,dw,time,direction,spread, Disp, intThresh, prevYaw, prevCoeffMD, prevCoeffRE, prevCoeffIM);

end
